simulink model "vRTHS_MDOF_SimRT2014a"  (R2014a)
settings: Solver=ode4  StartTime=0.0  StopTime=tend  FixedStep=dt_rths  RelTol=1e-3
values from neighbouring files (symbols this model uses):
  a1_beta0 = 2.1283e+13    (= 21283000000000)    [F1_input_file.m]
  a2 = 4.2297e+06    (= 4229700)    [F1_input_file.m]
  a3 = 3.3        + 1.3   * nom *randn(1,1)    [F1_input_file.m]
  A_ns = [     zeros(n) eye(n) ... (first row only)    [F1_input_file.m]
  B_ns = [     zeros(n,1)      zeros(n) ... (first row only)    [F1_input_file.m]
  beta1 = 425        + 3.3   * nom *randn(1,1)    [F1_input_file.m]
  beta2 = 9.9976e+04 + 3.3e3 * nom *randn(1,1)    [F1_input_file.m]
  C_ns = [     eye(n)              zeros(n) ... (first row only)    [F1_input_file.m]
  CE = zeros(n)    [F1_input_file.m]
  D_ns = [     zeros(n,1)            zeros(n) ... (first row only)    [F1_input_file.m]
  dt_rths = 0.000244140625    [Plant.mat]    (also in RUN_vRTHS_demo_new.m)
  E_sw = 1    [F1_input_file.m]
  eq_intensity = .4    (= 0.4)    [F1_input_file.m]
  gain = 1.0261    [F1_input_file.m]
  Gsnsr_DT = 1    [F1_input_file.m]
  Gsnsr_FT = 1    [F1_input_file.m]
  KE = zeros(n)    [F1_input_file.m]
  ME = ME*1.3    [F1_Modifications.m]    (also in F1_input_file.m = zeros(n))
  Seed_snr = rng(seed)    [F1_input_file.m]
  tend = 90    [F1_input_file.m]
libraries: simulink x3, rtwinlib x1
settings Model: CovSFcnEnable=on  Creator=IISL_0175  LastModifiedBy=Sandra
settings DataIOCC: LimitDataPoints=off  SaveFormat=StructureWithTime
settings DebuggingCC: MergeDetectMultiDrivingBlocksExec=error  SolverPrmCheckMsg=none  InheritedTsInSrcMsg=none  FrameProcessingCompatibilityMsg=error
settings HardwareCC: ProdBitPerPointer=64  ProdLargestAtomicFloat=Float  ProdIntDivRoundTo=Zero  ProdEndianess=LittleEndian  ProdHWDeviceType=Specified
settings ModelReferenceCC: PropagateSignalLabelsOutOfModel=on

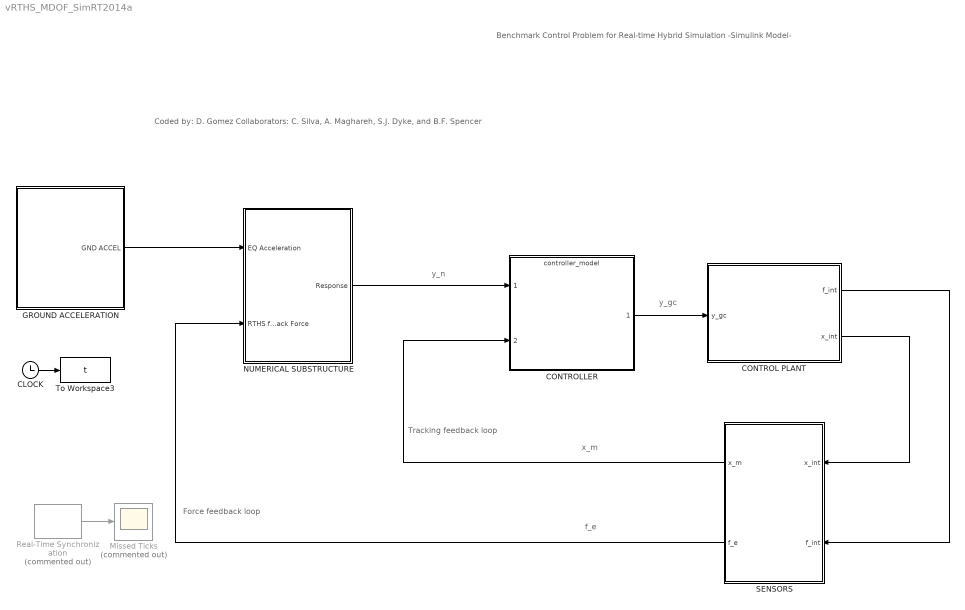
== system vRTHS_MDOF_SimRT2014a ==
  note: Force
      | feedback loop
  note: Benchmark Control Problem for Real-time Hybrid Simulation
      | -Simulink Model-
  note: Coded by: D. Gomez
      | Collaborators: C. Silva, A. Maghareh, S.J. Dyke, and B.F. Spencer
  note: Tracking feedback loop
  note: y_n
  note: y_gc
  note: f_e
  note: x_m
  CLOCK : Clock
  CONTROL PLANT : Subsystem
      mask Display: image(imread('PlantSW2.PNG'));
  CONTROLLER : ModelReference  ModelNameDialog=controller_model.slx  SimulationMode=Normal  ModelReferenceVersion=1.7
  GROUND ACCELERATION : Subsystem
  Missed Ticks : Scope  Commented=on
      settings: TimeRange=10  MaxDataPoints=5000  SaveToWorkspace=off  YMin=-51.75  YMax=465.75  SampleTime=-1  DataFormat=Structure
  NUMERICAL SUBSTRUCTURE : Subsystem
      mask Display: image(imread('Num_sub.png'));
  Real-Time Synchronization : rtwinlib/Real-Time Synchronization  Commented=on  SampleTime=dt_rths  MaxMissedTicks=10000  ShowMissedTicks=on  YieldWhenWaiting=off
  SENSORS : Subsystem
  To Workspace3 : ToWorkspace  VariableName=t  SampleTime=-1
  wires:
  CLOCK/1 -> To Workspace3/1
  CONTROL PLANT/2(x_int) -> SENSORS/1(x_int)
  SENSORS/2("f_e ") -> NUMERICAL SUBSTRUCTURE/2(RTHS feedback Force)
  CONTROLLER/1 -> CONTROL PLANT/1(y_gc)
  NUMERICAL SUBSTRUCTURE/1(Response) -> CONTROLLER/1
  Real-Time Synchronization/1 -> Missed Ticks/1
  SENSORS/1(x_m) -> CONTROLLER/2
  GROUND ACCELERATION/1(GND ACCEL) -> NUMERICAL SUBSTRUCTURE/1(EQ Acceleration)
  CONTROL PLANT/1(f_int) -> SENSORS/2(f_int)

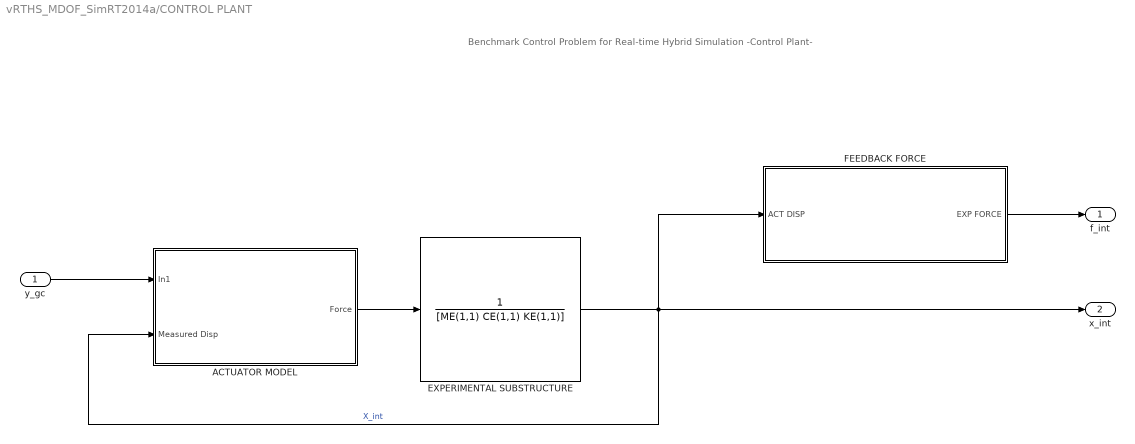
== system vRTHS_MDOF_SimRT2014a/CONTROL PLANT ==
  note: Benchmark Control Problem for Real-time Hybrid Simulation
      | -Control Plant-
  y_gc : Inport
  ACTUATOR MODEL : Subsystem
      mask Display: image(imread('ActuatorSW2.PNG'));
  EXPERIMENTAL SUBSTRUCTURE : TransferFcn  Numerator=1  Denominator=[ME(1,1) CE(1,1) KE(1,1)]
      mask Display: image(imread('ESSW2.PNG'));
  FEEDBACK FORCE : Subsystem
  f_int : Outport
  x_int : Outport  Port=2
  wires:
  y_gc/1 -> ACTUATOR MODEL/1(In1)
  EXPERIMENTAL SUBSTRUCTURE/1 -> FEEDBACK FORCE/1(ACT DISP), x_int/1, ACTUATOR MODEL/2(Measured Disp)  "X_int"
  ACTUATOR MODEL/1(Force) -> EXPERIMENTAL SUBSTRUCTURE/1
  FEEDBACK FORCE/1(EXP FORCE) -> f_int/1

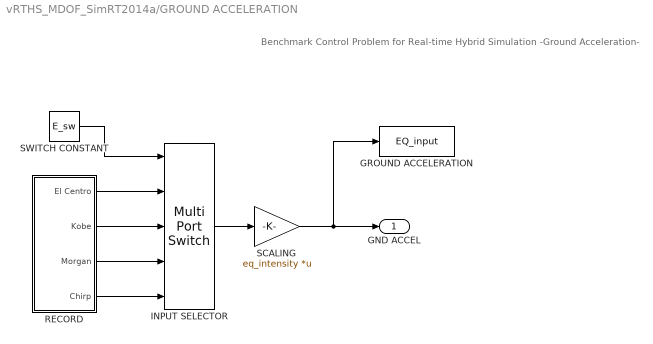
== system vRTHS_MDOF_SimRT2014a/GROUND ACCELERATION ==
  note: Benchmark Control Problem for Real-time Hybrid Simulation
      | -Ground Acceleration-
  GROUND ACCELERATION : ToWorkspace  VariableName=EQ_input  SampleTime=-1
  INPUT SELECTOR : MultiPortSwitch  Inputs=4
  "RECORD " : Subsystem
  SCALING : Gain  Gain=eq_intensity  Multiplication=Matrix(K*u)
  SWITCH CONSTANT : Constant  Value=E_sw
  GND ACCEL : Outport
  wires:
  INPUT SELECTOR/1 -> SCALING/1
  SWITCH CONSTANT/1 -> INPUT SELECTOR/1
  "RECORD "/1(El Centro) -> INPUT SELECTOR/2
  "RECORD "/2(Kobe) -> INPUT SELECTOR/3
  "RECORD "/3(Morgan) -> INPUT SELECTOR/4
  SCALING/1 -> GROUND ACCELERATION/1, GND ACCEL/1
  "RECORD "/4(Chirp) -> INPUT SELECTOR/5

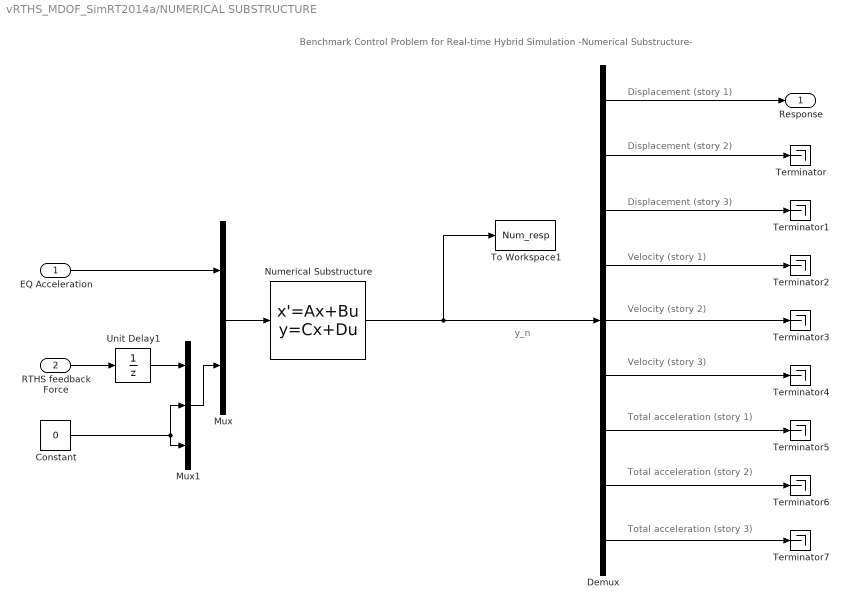
== system vRTHS_MDOF_SimRT2014a/NUMERICAL SUBSTRUCTURE ==
  note: y_n
  note: Benchmark Control Problem for Real-time Hybrid Simulation
      | -Numerical Substructure-
  note: Velocity (story 3)
  note: Displacement (story 3)
  note: Displacement (story 1)
  note: Total acceleration (story 1)
  note: Velocity (story 1)
  note: Velocity (story 2)
  note: Total acceleration (story 3)
  note: Displacement (story 2)
  note: Total acceleration (story 2)
  EQ Acceleration : Inport
  RTHS feedback Force : Inport  Port=2
  Constant : Constant  Value=0
  Demux : Demux  Outputs=9
  Mux : Mux  Inputs=2
  Mux1 : Mux  Inputs=3
  Numerical Substructure : StateSpace  A=A_ns  B=B_ns  C=C_ns  D=D_ns  X0=0
  Terminator{,1..7} (8 alike) : Terminator
  To Workspace1 : ToWorkspace  VariableName=Num_resp  SaveFormat=Timeseries  SampleTime=-1
  Unit Delay1 : UnitDelay  SampleTime=-1
  Response : Outport
  wires:
  Mux/1 -> Numerical Substructure/1
  EQ Acceleration/1 -> Mux/1
  RTHS feedback Force/1 -> Unit Delay1/1
  Numerical Substructure/1 -> To Workspace1/1, Demux/1
  Demux/2 -> Terminator/1
  Demux/7 -> Terminator5/1
  Demux/8 -> Terminator6/1
  Demux/9 -> Terminator7/1
  Demux/4 -> Terminator2/1
  Demux/6 -> Terminator4/1
  Demux/5 -> Terminator3/1
  Demux/1 -> Response/1
  Demux/3 -> Terminator1/1
  Constant/1 -> Mux1/2, Mux1/3
  Mux1/1 -> Mux/2
  Unit Delay1/1 -> Mux1/1

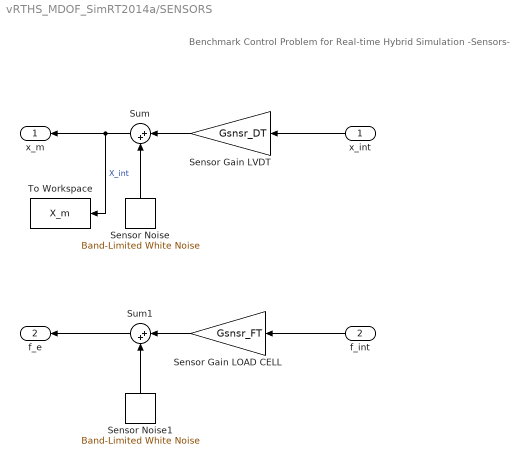
== system vRTHS_MDOF_SimRT2014a/SENSORS ==
  note: Benchmark Control Problem for Real-time Hybrid Simulation
      | -Sensors-
  x_int : Inport
  f_int : Inport  Port=2
  Sensor Noise : simulink/Sources/Band-Limited White Noise  Cov=rms_noise_DT  Ts=dt_rths  seed=double(Seed_snr.Seed)
  Sensor Noise1 : simulink/Sources/Band-Limited White Noise  Cov=rms_noise_FT  Ts=dt_rths  seed=double(Seed_snr.Seed)
  Sensor Gain LVDT : Gain  Gain=Gsnsr_DT  SaturateOnIntegerOverflow=on  OutDataTypeStr=Inherit: Same as input  ParamDataTypeStr=Inherit: Same as input
  Sensor Gain LOAD CELL : Gain  Gain=Gsnsr_FT  SaturateOnIntegerOverflow=on  OutDataTypeStr=Inherit: Same as input  ParamDataTypeStr=Inherit: Same as input
  Sum : Sum  Inputs=|++  SaturateOnIntegerOverflow=on  InputSameDT=on  OutDataTypeStr=Inherit: Same as first input
  Sum1 : Sum  Inputs=|++  SaturateOnIntegerOverflow=on  InputSameDT=on  OutDataTypeStr=Inherit: Same as first input
  To Workspace : ToWorkspace  VariableName=X_m  SaveFormat=Timeseries  SampleTime=-1
  x_m : Outport
  "f_e " : Outport  Port=2
  wires:
  Sensor Gain LVDT/1 -> Sum/1
  Sensor Noise/1 -> Sum/2
  x_int/1 -> Sensor Gain LVDT/1
  Sensor Gain LOAD CELL/1 -> Sum1/1
  Sum1/1 -> "f_e "/1
  Sensor Noise1/1 -> Sum1/2
  f_int/1 -> Sensor Gain LOAD CELL/1
  Sum/1 -> x_m/1, To Workspace/1  "X_int"

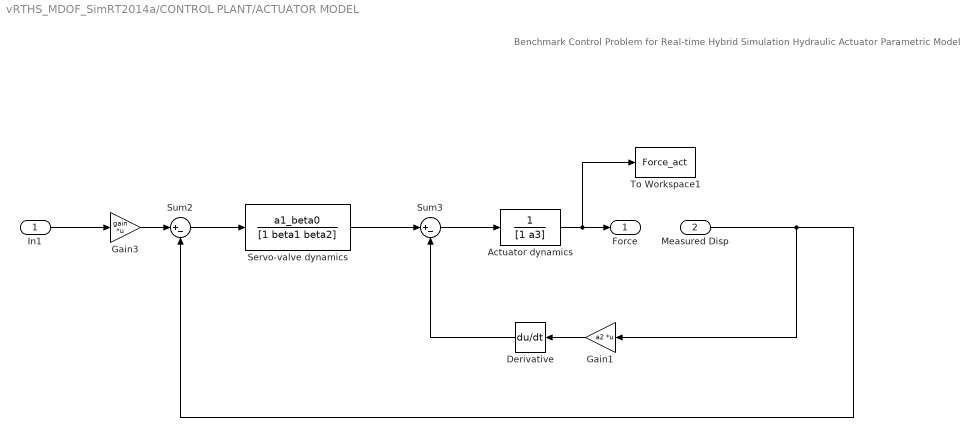
== system vRTHS_MDOF_SimRT2014a/CONTROL PLANT/ACTUATOR MODEL ==
  note: Benchmark Control Problem for Real-time Hybrid Simulation
      | Hydraulic Actuator Parametric Model
  In1 : Inport
  Measured Disp : Inport  Port=2
  Actuator dynamics : TransferFcn  Numerator=1  Denominator=[1 a3]
  Derivative : Derivative
  Gain1 : Gain  Gain=a2  Multiplication=Matrix(K*u)
  Gain3 : Gain  Gain=gain  Multiplication=Matrix(K*u)
  Servo-valve dynamics : TransferFcn  Numerator=a1_beta0  Denominator=[1 beta1 beta2]
  Sum2 : Sum  Inputs=|+-
  Sum3 : Sum  Inputs=|+-
  To Workspace1 : ToWorkspace  VariableName=Force_act  SaveFormat=Timeseries  SampleTime=-1
  Force : Outport
  wires:
  Gain3/1 -> Sum2/1
  Actuator dynamics/1 -> To Workspace1/1, Force/1
  Servo-valve dynamics/1 -> Sum3/1
  In1/1 -> Gain3/1
  Sum2/1 -> Servo-valve dynamics/1
  Gain1/1 -> Derivative/1
  Derivative/1 -> Sum3/2
  Sum3/1 -> Actuator dynamics/1
  Measured Disp/1 -> Sum2/2, Gain1/1

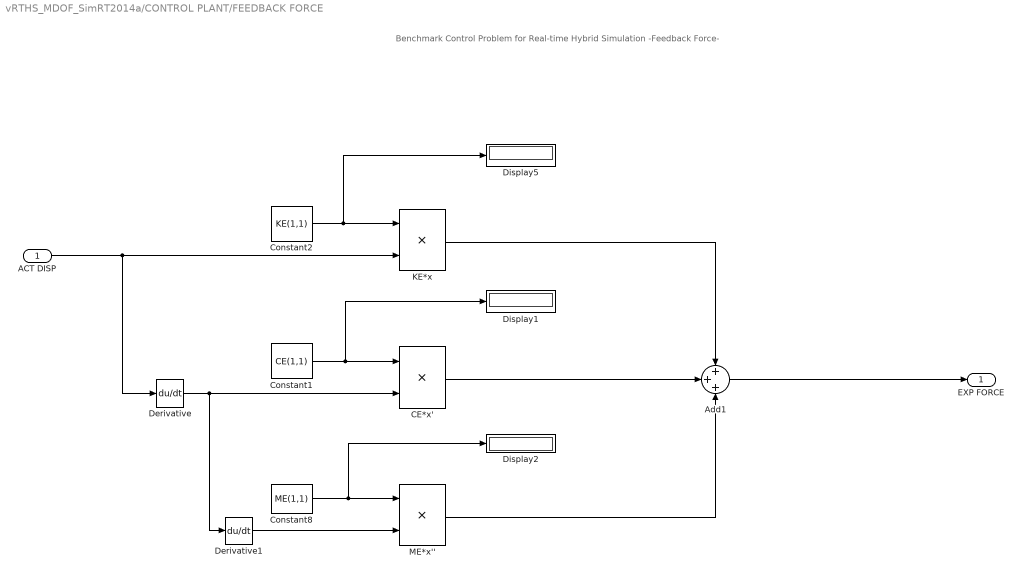
== system vRTHS_MDOF_SimRT2014a/CONTROL PLANT/FEEDBACK FORCE ==
  note: Benchmark Control Problem for Real-time Hybrid Simulation
      | -Feedback Force-
  ACT DISP : Inport
  Add1 : Sum  Inputs=+++
  CE*x' : Product  RndMeth=Zero
  Constant1 : Constant  Value=CE(1,1)  VectorParams1D=off
  Constant2 : Constant  Value=KE(1,1)  VectorParams1D=off
  Constant8 : Constant  Value=ME(1,1)  VectorParams1D=off
  Derivative : Derivative
  Derivative1 : Derivative
  Display1 : Display
  Display2 : Display
  Display5 : Display
  KE*x : Product  RndMeth=Zero
  ME*x'' : Product  RndMeth=Zero
  EXP FORCE : Outport
  wires:
  Constant1/1 -> Display1/1, CE*x'/1
  Constant8/1 -> Display2/1, ME*x''/1
  ACT DISP/1 -> KE*x/2, Derivative/1
  Derivative/1 -> CE*x'/2, Derivative1/1
  Derivative1/1 -> ME*x''/2
  Constant2/1 -> KE*x/1, Display5/1
  Add1/1 -> EXP FORCE/1
  KE*x/1 -> Add1/1
  CE*x'/1 -> Add1/2
  ME*x''/1 -> Add1/3

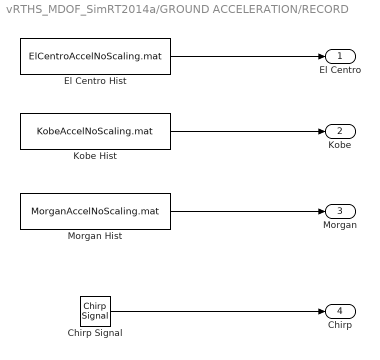
== system vRTHS_MDOF_SimRT2014a/GROUND ACCELERATION/RECORD  ==
  Chirp Signal : simulink/Sources/Chirp Signal  f1=f_ini  T=tend  f2=f_end
  El Centro Hist : FromFile  FileName=ElCentroAccelNoScaling.mat
  Kobe Hist : FromFile  FileName=KobeAccelNoScaling.mat
  Morgan Hist : FromFile  FileName=MorganAccelNoScaling.mat
  El Centro : Outport
  Kobe : Outport  Port=2
  Morgan : Outport  Port=3
  Chirp : Outport  Port=4
  wires:
  Morgan Hist/1 -> Morgan/1
  Kobe Hist/1 -> Kobe/1
  El Centro Hist/1 -> El Centro/1
  Chirp Signal/1 -> Chirp/1
